simulink model "orig_exp3_compound"  (R2023a)
settings: Solver=ode4  StartTime=0.0  StopTime=8  FixedStep=0.0005  RelTol=1e-3
settings Model: Creator=Anonymous  LastModifiedBy=Anonymous

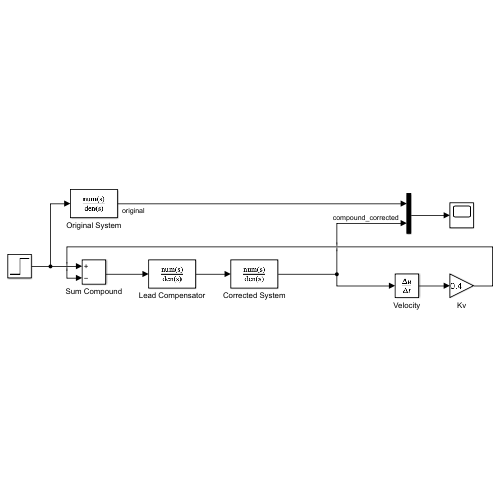
[thumbnail: Simulink's stored preview of the top-level diagram]
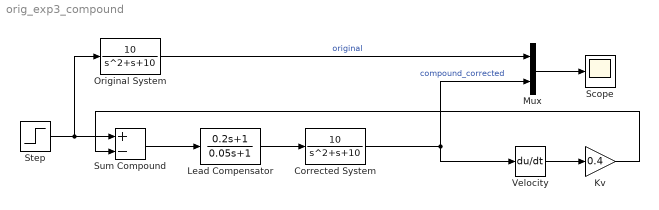
== system orig_exp3_compound ==
  Corrected System : TransferFcn  Numerator=10  Denominator=[1 1 10]
  Kv : Gain  Gain=0.4
  Lead Compensator : TransferFcn  Numerator=[0.2 1]  Denominator=[0.05 1]
  Mux : Mux  Inputs=2
  Original System : TransferFcn  Numerator=10  Denominator=[1 1 10]
  Scope : Scope
  Step : Step  Time=0  SampleTime=0
  Sum Compound : Sum  Inputs=+-
  Velocity : Derivative
  wires:
  Mux/1 -> Scope/1
  Kv/1 -> Sum Compound/2
  Velocity/1 -> Kv/1
  Corrected System/1 -> Mux/2, Velocity/1  "compound_corrected"
  Lead Compensator/1 -> Corrected System/1
  Sum Compound/1 -> Lead Compensator/1
  Original System/1 -> Mux/1  "original"
  Step/1 -> Sum Compound/1, Original System/1
